simulink subsystem "HydrostaticCVT"  (R2025a)
settings: Solver=VariableStepAuto  StartTime=0.0  StopTime=10.0  RelTol=1e-3
undefined symbols (not defined in the file): fluids, hydrostaticCVT
libraries: fl_lib x48, nesl_utility x21, SimscapeFluids_lib x10
(part 2 of 2)

== system HydrostaticCVT/Pipe A/p2 ==
  PS-Simulink Converter : nesl_utility/PS-Simulink Converter  PhysicalDomain=network_engine_domain  SubClassName=ps_output  LeftPortType=input  RightPortType=output  PseudoPeriodic=off  Frequencies=[]  VectorFormat=1-D array  Unit=bar  AffineConversion=off
  Pressure Sensor (IL) : fl_lib/Isothermal Liquid/Sensors/Pressure Sensor (IL)  pressure_measure=foundation.enum.pressure_measure.difference
      settings: InternalSimscapePortConfiguration="{\"Bottom\":[],\"Left\":[{\"id\":\"A\",\"label\":\"A\",\"type\":\"foundation.isothermal_liquid.isothermal_liquid\"}],\"Right\":[{\"id\":\"B\",\"label\":\"B\",\"type\":\"foundation.isothermal_liquid.isothermal_liquid\"},{\"id\":\"P\",\"label\":\"P\",\"type\":\"output\"}],\"Top\":[]}"
  Reservoir (IL)1 : fl_lib/Isothermal Liquid/Elements/Reservoir (IL)  reservoir_type=foundation.enum.constant_controlled.constant  pressure_spec=foundation.enum.pressure_spec.atmospheric  reservoir_pressure=0.101325 MPa
  A : PMIOPort  Side=Left
  " P" : Outport
  wires:
  PS-Simulink Converter/1 -> " P"/1
  connections:
  Pressure Sensor (IL)/LConn1 -- A/RConn1
  Reservoir (IL)1/LConn1 -- Pressure Sensor (IL)/RConn1
  PS-Simulink Converter/LConn1 -- Pressure Sensor (IL)/RConn2

== system HydrostaticCVT/Pipe A/p5 ==
  PS-Simulink Converter : nesl_utility/PS-Simulink Converter  PhysicalDomain=network_engine_domain  SubClassName=ps_output  LeftPortType=input  RightPortType=output  PseudoPeriodic=off  Frequencies=[]  VectorFormat=1-D array  Unit=bar  AffineConversion=off
  Pressure Sensor (IL) : fl_lib/Isothermal Liquid/Sensors/Pressure Sensor (IL)  pressure_measure=foundation.enum.pressure_measure.difference
      settings: InternalSimscapePortConfiguration="{\"Bottom\":[],\"Left\":[{\"id\":\"A\",\"label\":\"A\",\"type\":\"foundation.isothermal_liquid.isothermal_liquid\"}],\"Right\":[{\"id\":\"B\",\"label\":\"B\",\"type\":\"foundation.isothermal_liquid.isothermal_liquid\"},{\"id\":\"P\",\"label\":\"P\",\"type\":\"output\"}],\"Top\":[]}"
  Reservoir (IL)1 : fl_lib/Isothermal Liquid/Elements/Reservoir (IL)  reservoir_type=foundation.enum.constant_controlled.constant  pressure_spec=foundation.enum.pressure_spec.atmospheric  reservoir_pressure=0.101325 MPa
  A : PMIOPort  Side=Left
  " P" : Outport
  wires:
  PS-Simulink Converter/1 -> " P"/1
  connections:
  PS-Simulink Converter/LConn1 -- Pressure Sensor (IL)/RConn2
  Reservoir (IL)1/LConn1 -- Pressure Sensor (IL)/RConn1
  Pressure Sensor (IL)/LConn1 -- A/RConn1

== system HydrostaticCVT/Pipe B/Q1 ==
  Flow Rate Sensor (IL) : fl_lib/Isothermal Liquid/Sensors/Flow Rate Sensor (IL)  sensor_type=foundation.enum.mass_volumetric_sensor.mass_volumetric
      settings: InternalSimscapePortConfiguration="{\"Bottom\":[],\"Left\":[{\"id\":\"A\",\"label\":\"A\",\"type\":\"foundation.isothermal_liquid.isothermal_liquid\"}],\"Right\":[{\"id\":\"B\",\"label\":\"B\",\"type\":\"foundation.isothermal_liquid.isothermal_liquid\"},{\"id\":\"M\",\"label\":\"M\",\"type\":\"output\"},{\"id\":\"V\",\"label\":\"V\",\"type\":\"output\"}],\"Top\":[]}"
  PS Terminator : fl_lib/Physical Signals/Sinks/PS Terminator
  PS-Simulink Converter : nesl_utility/PS-Simulink Converter  PhysicalDomain=network_engine_domain  SubClassName=ps_output  LeftPortType=input  RightPortType=output  PseudoPeriodic=off  Frequencies=[]  VectorFormat=1-D array  Unit=m^3/s  AffineConversion=off
  A : PMIOPort  Side=Left
  B : PMIOPort  Port=2  Side=Right
  Q : Outport
  wires:
  PS-Simulink Converter/1 -> Q/1
  connections:
  Flow Rate Sensor (IL)/RConn2 -- PS Terminator/LConn1
  Flow Rate Sensor (IL)/RConn3 -- PS-Simulink Converter/LConn1
  Flow Rate Sensor (IL)/RConn1 -- B/RConn1
  A/RConn1 -- Flow Rate Sensor (IL)/LConn1

== system HydrostaticCVT/Pipe B/Q3 ==
  Flow Rate Sensor (IL) : fl_lib/Isothermal Liquid/Sensors/Flow Rate Sensor (IL)  sensor_type=foundation.enum.mass_volumetric_sensor.mass_volumetric
      settings: InternalSimscapePortConfiguration="{\"Bottom\":[],\"Left\":[{\"id\":\"A\",\"label\":\"A\",\"type\":\"foundation.isothermal_liquid.isothermal_liquid\"}],\"Right\":[{\"id\":\"B\",\"label\":\"B\",\"type\":\"foundation.isothermal_liquid.isothermal_liquid\"},{\"id\":\"M\",\"label\":\"M\",\"type\":\"output\"},{\"id\":\"V\",\"label\":\"V\",\"type\":\"output\"}],\"Top\":[]}"
  PS Terminator : fl_lib/Physical Signals/Sinks/PS Terminator
  PS-Simulink Converter : nesl_utility/PS-Simulink Converter  PhysicalDomain=network_engine_domain  SubClassName=ps_output  LeftPortType=input  RightPortType=output  PseudoPeriodic=off  Frequencies=[]  VectorFormat=1-D array  Unit=m^3/s  AffineConversion=off
  A : PMIOPort  Side=Left
  B : PMIOPort  Port=2  Side=Right
  Q : Outport
  wires:
  PS-Simulink Converter/1 -> Q/1
  connections:
  A/RConn1 -- Flow Rate Sensor (IL)/LConn1
  Flow Rate Sensor (IL)/RConn1 -- B/RConn1
  Flow Rate Sensor (IL)/RConn3 -- PS-Simulink Converter/LConn1
  Flow Rate Sensor (IL)/RConn2 -- PS Terminator/LConn1

== system HydrostaticCVT/Pipe B/p2 ==
  PS-Simulink Converter : nesl_utility/PS-Simulink Converter  PhysicalDomain=network_engine_domain  SubClassName=ps_output  LeftPortType=input  RightPortType=output  PseudoPeriodic=off  Frequencies=[]  VectorFormat=1-D array  Unit=bar  AffineConversion=off
  Pressure Sensor (IL) : fl_lib/Isothermal Liquid/Sensors/Pressure Sensor (IL)  pressure_measure=foundation.enum.pressure_measure.difference
      settings: InternalSimscapePortConfiguration="{\"Bottom\":[],\"Left\":[{\"id\":\"A\",\"label\":\"A\",\"type\":\"foundation.isothermal_liquid.isothermal_liquid\"}],\"Right\":[{\"id\":\"B\",\"label\":\"B\",\"type\":\"foundation.isothermal_liquid.isothermal_liquid\"},{\"id\":\"P\",\"label\":\"P\",\"type\":\"output\"}],\"Top\":[]}"
  Reservoir (IL)1 : fl_lib/Isothermal Liquid/Elements/Reservoir (IL)  reservoir_type=foundation.enum.constant_controlled.constant  pressure_spec=foundation.enum.pressure_spec.atmospheric  reservoir_pressure=0.101325 MPa
  A : PMIOPort  Side=Left
  " P" : Outport
  wires:
  PS-Simulink Converter/1 -> " P"/1
  connections:
  Pressure Sensor (IL)/LConn1 -- A/RConn1
  Reservoir (IL)1/LConn1 -- Pressure Sensor (IL)/RConn1
  PS-Simulink Converter/LConn1 -- Pressure Sensor (IL)/RConn2

== system HydrostaticCVT/Pipe B/p5 ==
  PS-Simulink Converter : nesl_utility/PS-Simulink Converter  PhysicalDomain=network_engine_domain  SubClassName=ps_output  LeftPortType=input  RightPortType=output  PseudoPeriodic=off  Frequencies=[]  VectorFormat=1-D array  Unit=bar  AffineConversion=off
  Pressure Sensor (IL) : fl_lib/Isothermal Liquid/Sensors/Pressure Sensor (IL)  pressure_measure=foundation.enum.pressure_measure.difference
      settings: InternalSimscapePortConfiguration="{\"Bottom\":[],\"Left\":[{\"id\":\"A\",\"label\":\"A\",\"type\":\"foundation.isothermal_liquid.isothermal_liquid\"}],\"Right\":[{\"id\":\"B\",\"label\":\"B\",\"type\":\"foundation.isothermal_liquid.isothermal_liquid\"},{\"id\":\"P\",\"label\":\"P\",\"type\":\"output\"}],\"Top\":[]}"
  Reservoir (IL)1 : fl_lib/Isothermal Liquid/Elements/Reservoir (IL)  reservoir_type=foundation.enum.constant_controlled.constant  pressure_spec=foundation.enum.pressure_spec.atmospheric  reservoir_pressure=0.101325 MPa
  A : PMIOPort  Side=Left
  " P" : Outport
  wires:
  PS-Simulink Converter/1 -> " P"/1
  connections:
  PS-Simulink Converter/LConn1 -- Pressure Sensor (IL)/RConn2
  Reservoir (IL)1/LConn1 -- Pressure Sensor (IL)/RConn1
  Pressure Sensor (IL)/LConn1 -- A/RConn1

== system HydrostaticCVT/Rear Motor/Q5 ==
  Flow Rate Sensor (IL) : fl_lib/Isothermal Liquid/Sensors/Flow Rate Sensor (IL)  sensor_type=foundation.enum.mass_volumetric_sensor.mass_volumetric
      settings: InternalSimscapePortConfiguration="{\"Bottom\":[],\"Left\":[{\"id\":\"A\",\"label\":\"A\",\"type\":\"foundation.isothermal_liquid.isothermal_liquid\"}],\"Right\":[{\"id\":\"B\",\"label\":\"B\",\"type\":\"foundation.isothermal_liquid.isothermal_liquid\"},{\"id\":\"M\",\"label\":\"M\",\"type\":\"output\"},{\"id\":\"V\",\"label\":\"V\",\"type\":\"output\"}],\"Top\":[]}"
  PS Terminator : fl_lib/Physical Signals/Sinks/PS Terminator
  PS-Simulink Converter : nesl_utility/PS-Simulink Converter  PhysicalDomain=network_engine_domain  SubClassName=ps_output  LeftPortType=input  RightPortType=output  PseudoPeriodic=off  Frequencies=[]  VectorFormat=1-D array  Unit=m^3/s  AffineConversion=off
  A : PMIOPort  Side=Left
  B : PMIOPort  Port=2  Side=Right
  Q : Outport
  wires:
  PS-Simulink Converter/1 -> Q/1
  connections:
  A/RConn1 -- Flow Rate Sensor (IL)/LConn1
  Flow Rate Sensor (IL)/RConn1 -- B/RConn1
  Flow Rate Sensor (IL)/RConn3 -- PS-Simulink Converter/LConn1
  Flow Rate Sensor (IL)/RConn2 -- PS Terminator/LConn1

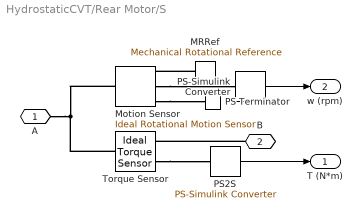
== system HydrostaticCVT/Rear Motor/S ==
  MRRef : fl_lib/Mechanical/Rotational Elements/Mechanical Rotational Reference
  Motion Sensor : fl_lib/Mechanical/Mechanical Sensors/Ideal Rotational Motion Sensor  reference=foundation.enum.MeasurementReference.difference  acceleration_port=false  velocity_port=true  position_port=true  wrap_angle=simscape.enum.onoff.off  offset=0 rad
  PS Terminator : fl_lib/Physical Signals/Sinks/PS Terminator
  PS-Simulink Converter : nesl_utility/PS-Simulink Converter  PhysicalDomain=network_engine_domain  SubClassName=ps_output  LeftPortType=input  RightPortType=output  PseudoPeriodic=off  Frequencies=[]  VectorFormat=1-D array  Unit=rpm  AffineConversion=off
  PS2S : nesl_utility/PS-Simulink Converter  PhysicalDomain=network_engine_domain  SubClassName=ps_output  LeftPortType=input  RightPortType=output  PseudoPeriodic=off  Frequencies=[]  VectorFormat=1-D array  Unit=N*m  AffineConversion=off
  Torque Sensor : fl_lib/Mechanical/Mechanical Sensors/Ideal Torque Sensor
  A : PMIOPort  Side=Left
  B : PMIOPort  Port=2  Side=Right
  T (N*m) : Outport
  w (rpm) : Outport  Port=2
  wires:
  PS-Simulink Converter/1 -> w (rpm)/1
  PS2S/1 -> T (N*m)/1
  connections:
  Motion Sensor/RConn3 -- PS Terminator/LConn1
  B/RConn1 -- Torque Sensor/RConn1
  Torque Sensor/RConn2 -- PS2S/LConn1
  MRRef/LConn1 -- Motion Sensor/RConn1
  Motion Sensor/RConn2 -- PS-Simulink Converter/LConn1
  Motion Sensor/LConn1 -- A/RConn1 -- Torque Sensor/LConn1

== system HydrostaticCVT/Relief Valve A/Q8 ==
  Flow Rate Sensor (IL) : fl_lib/Isothermal Liquid/Sensors/Flow Rate Sensor (IL)  sensor_type=foundation.enum.mass_volumetric_sensor.mass_volumetric
      settings: InternalSimscapePortConfiguration="{\"Bottom\":[],\"Left\":[{\"id\":\"A\",\"label\":\"A\",\"type\":\"foundation.isothermal_liquid.isothermal_liquid\"}],\"Right\":[{\"id\":\"B\",\"label\":\"B\",\"type\":\"foundation.isothermal_liquid.isothermal_liquid\"},{\"id\":\"M\",\"label\":\"M\",\"type\":\"output\"},{\"id\":\"V\",\"label\":\"V\",\"type\":\"output\"}],\"Top\":[]}"
  PS Terminator : fl_lib/Physical Signals/Sinks/PS Terminator
  PS-Simulink Converter : nesl_utility/PS-Simulink Converter  PhysicalDomain=network_engine_domain  SubClassName=ps_output  LeftPortType=input  RightPortType=output  PseudoPeriodic=off  Frequencies=[]  VectorFormat=1-D array  Unit=m^3/s  AffineConversion=off
  A : PMIOPort  Side=Left
  B : PMIOPort  Port=2  Side=Right
  Q : Outport
  wires:
  PS-Simulink Converter/1 -> Q/1
  connections:
  Flow Rate Sensor (IL)/RConn2 -- PS Terminator/LConn1
  Flow Rate Sensor (IL)/RConn3 -- PS-Simulink Converter/LConn1
  Flow Rate Sensor (IL)/RConn1 -- B/RConn1
  A/RConn1 -- Flow Rate Sensor (IL)/LConn1

== system HydrostaticCVT/Relief Valve B/Q4 ==
  Flow Rate Sensor (IL) : fl_lib/Isothermal Liquid/Sensors/Flow Rate Sensor (IL)  sensor_type=foundation.enum.mass_volumetric_sensor.mass_volumetric
      settings: InternalSimscapePortConfiguration="{\"Bottom\":[],\"Left\":[{\"id\":\"A\",\"label\":\"A\",\"type\":\"foundation.isothermal_liquid.isothermal_liquid\"}],\"Right\":[{\"id\":\"B\",\"label\":\"B\",\"type\":\"foundation.isothermal_liquid.isothermal_liquid\"},{\"id\":\"M\",\"label\":\"M\",\"type\":\"output\"},{\"id\":\"V\",\"label\":\"V\",\"type\":\"output\"}],\"Top\":[]}"
  PS Terminator : fl_lib/Physical Signals/Sinks/PS Terminator
  PS-Simulink Converter : nesl_utility/PS-Simulink Converter  PhysicalDomain=network_engine_domain  SubClassName=ps_output  LeftPortType=input  RightPortType=output  PseudoPeriodic=off  Frequencies=[]  VectorFormat=1-D array  Unit=m^3/s  AffineConversion=off
  A : PMIOPort  Side=Left
  B : PMIOPort  Port=2  Side=Right
  Q : Outport
  wires:
  PS-Simulink Converter/1 -> Q/1
  connections:
  A/RConn1 -- Flow Rate Sensor (IL)/LConn1
  Flow Rate Sensor (IL)/RConn1 -- B/RConn1
  Flow Rate Sensor (IL)/RConn3 -- PS-Simulink Converter/LConn1
  Flow Rate Sensor (IL)/RConn2 -- PS Terminator/LConn1
